simulink model "UHG_PID_control"  (R2023a)
settings: Solver=VariableStepAuto  StartTime=0.0  StopTime=30  RelTol=1e-3
settings Model: Creator=tshintai  LastModifiedBy=tshintai
settings SolverCC: AlgebraicLoopSolver=TrustRegion
settings OptimizationCC: ReuseModelBlockBuffer=off
settings DebuggingCC: UnconnectedInputMsg=warning  UnconnectedOutputMsg=warning  UnconnectedLineMsg=warning
settings ModelReferenceCC: EnableRefExpFcnMdlSchedulingChecks=on
settings RTWCC: DLArmComputeVersion=19.05

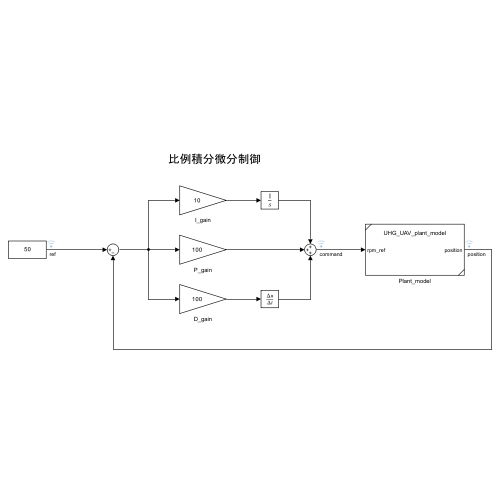
[thumbnail: Simulink's stored preview of the top-level diagram]
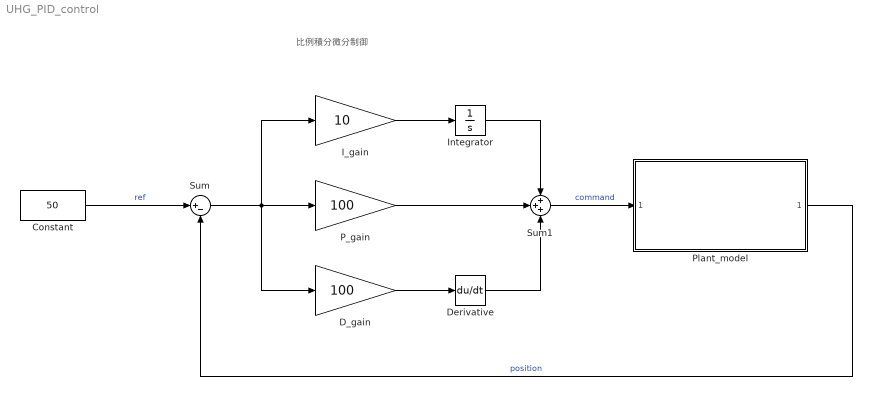
== system UHG_PID_control ==
  note: 比例積分微分制御
  Constant : Constant  Value=50
  D_gain : Gain  Gain=100
  Derivative : Derivative
  I_gain : Gain  Gain=10
  Integrator : Integrator
  P_gain : Gain  Gain=100
  Plant_model : Subsystem  ReferencedSubsystem=UHG_UAV_plant_model
  Sum : Sum  Inputs=|+-
  Sum1 : Sum  Inputs=+++
  wires:
  P_gain/1 -> Sum1/2
  Sum/1 -> D_gain/1, I_gain/1, P_gain/1
  Constant/1 -> Sum/1  "ref"
  Plant_model/1 -> Sum/2  "position"
  I_gain/1 -> Integrator/1
  Sum1/1 -> Plant_model/1  "command"
  Integrator/1 -> Sum1/1
  D_gain/1 -> Derivative/1
  Derivative/1 -> Sum1/3
